simulink model "canard_sim"  (R2026b)
settings: Solver=VariableStepAuto
values from neighbouring files (symbols this model uses):
  boosterCurve = thrustCurve("Data/Cesaroni_2856L910-P.csv")    [TestRocketSetup.m]
  boosterISP = 223    [Full_Rocket_Constants.m]    (also in TestRocketSetup.m = 229)
  InitialMass = SustainerWetMass + BoosterWetMass    (= 57.8)    [Full_Rocket_Constants.m]
  SeparationMass = BoosterDryMass    (= 9.59)    [Full_Rocket_Constants.m]
  stack_t_cg = sus_t_cg(before_sep)    [Full_Rocket_Constants.m]
  stack_x_cg = sus_x_cg(before_sep)    [Full_Rocket_Constants.m]
  Sustainer_Length = 0.381+0.317+1.19    (= 1.888)    [Full_Rocket_Constants.m]
  sustainerISP = 189    [Full_Rocket_Constants.m]
  t_sep = 4.997    [Full_Rocket_Constants.m]
undefined symbols (not defined in the file or in its folder): Stage_Tol, sustainerCurve
libraries: aerolibasang x2, aerolibwind2 x2, aerolibanim x1, aerolibatmos2 x1
settings Model: Creator=linda  LastModifiedBy=linda
settings RTWCC: GPUComputeCapability=5.0

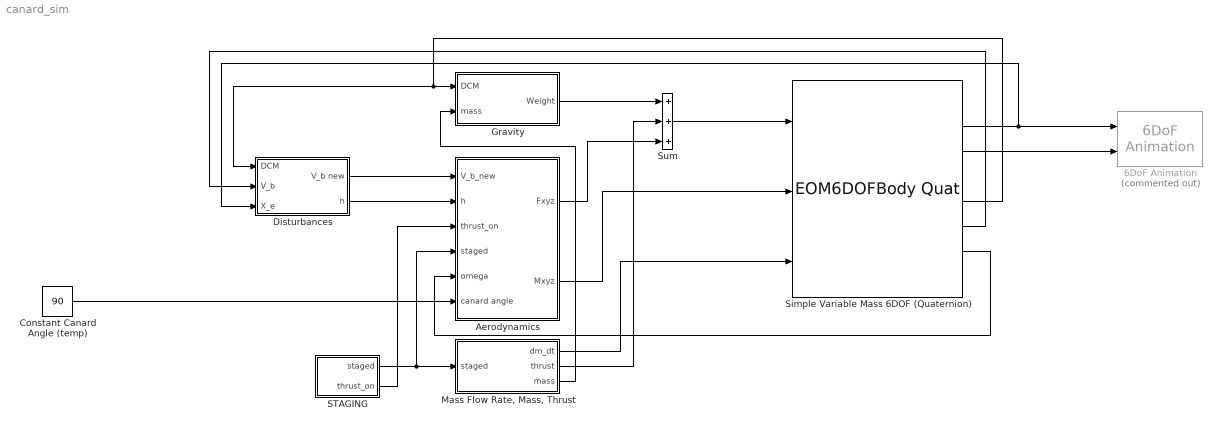
== system canard_sim ==
  6DoF Animation : aerolibanim/6DoF Animation  Commented=on  u1=[-4000 4000 -2000 2000 -5000000 4000000]  u2=0.1  u3=2  u4=[-1000 0 -1000]  u5=Fly alongside  u6=[40 5 -40]  u7=10  u8=on
  Aerodynamics : Subsystem
  Constant Canard Angle (temp) : Constant  Value=90
  Disturbances : Subsystem
  Gravity : Subsystem
  "Mass Flow Rate, Mass, Thrust" : Subsystem
  STAGING : Subsystem
  Simple Variable Mass 6DOF (Quaternion) : EOM6DOFBodyQuat  mtype=Simple Variable
  Sum : Sum  Inputs=+++
  wires:
  Aerodynamics/2(Mxyz) -> Simple Variable Mass 6DOF (Quaternion)/2
  Aerodynamics/1(Fxyz) -> Sum/3
  Sum/1 -> Simple Variable Mass 6DOF (Quaternion)/1
  "Mass Flow Rate, Mass, Thrust"/1(dm_dt) -> Simple Variable Mass 6DOF (Quaternion)/3
  Gravity/1(Weight) -> Sum/1
  "Mass Flow Rate, Mass, Thrust"/2(thrust) -> Sum/2
  Simple Variable Mass 6DOF (Quaternion)/3 -> 6DoF Animation/2
  Simple Variable Mass 6DOF (Quaternion)/2 -> 6DoF Animation/1, Disturbances/3(X_e)
  "Mass Flow Rate, Mass, Thrust"/3(mass) -> Gravity/2(mass)
  Simple Variable Mass 6DOF (Quaternion)/5 -> Disturbances/1(DCM), Gravity/1(DCM)
  Simple Variable Mass 6DOF (Quaternion)/6 -> Disturbances/2(V_b)
  Disturbances/2(h) -> Aerodynamics/2(h)
  STAGING/1(staged) -> "Mass Flow Rate, Mass, Thrust"/1(staged), Aerodynamics/4(staged)
  Disturbances/1(V_b new) -> Aerodynamics/1(V_b_new)
  STAGING/2(thrust_on) -> Aerodynamics/3(thrust_on)
  Simple Variable Mass 6DOF (Quaternion)/7 -> Aerodynamics/5(omega)
  Constant Canard Angle (temp)/1 -> Aerodynamics/6(canard angle)

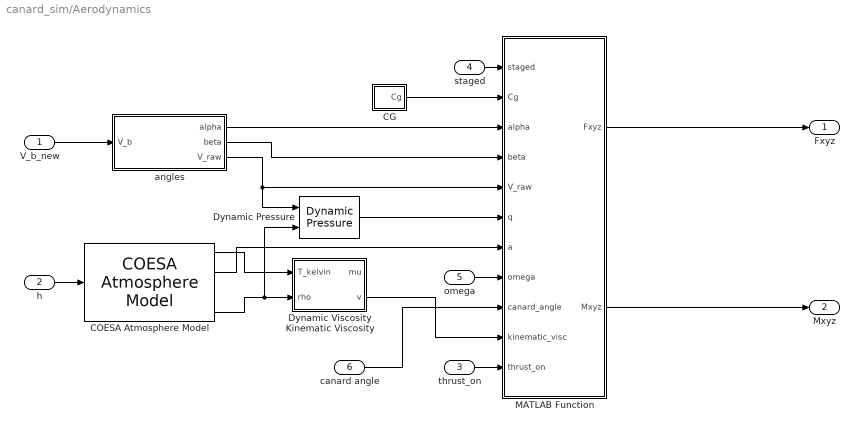
== system canard_sim/Aerodynamics ==
  V_b_new : Inport
  h : Inport  Port=2
  thrust_on : Inport  Port=3
  staged : Inport  Port=4
  omega : Inport  Port=5
  canard angle : Inport  Port=6
  CG : Subsystem
  COESA Atmosphere Model : aerolibatmos2/COESA Atmosphere Model  units=Metric (MKS)  spec=1976 COESA-extended U.S. Standard Atmosphere  model=Profile  profile_var=High temperature  profile_percent=1%  profile_alt=5 km (16404 ft)  envelope_var=High temperature  envelope_percent=1%  action=Warning
  Dynamic Pressure : aerolibasang/Dynamic Pressure
  Dynamic Viscosity Kinematic Viscosity : MATLAB Function  TreatAsAtomicUnit=on
  MATLAB Function : MATLAB Function  TreatAsAtomicUnit=on
  angles : MATLAB Function  TreatAsAtomicUnit=on
  Fxyz : Outport
  Mxyz : Outport  Port=2
  wires:
  COESA Atmosphere Model/1 -> Dynamic Viscosity Kinematic Viscosity/1(T_kelvin)
  COESA Atmosphere Model/4 -> Dynamic Viscosity Kinematic Viscosity/2(rho), Dynamic Pressure/2
  Dynamic Viscosity Kinematic Viscosity/2(v) -> MATLAB Function/10(kinematic_visc)
  Dynamic Pressure/1 -> MATLAB Function/6(q)
  COESA Atmosphere Model/2 -> MATLAB Function/7(a)
  h/1 -> COESA Atmosphere Model/1
  MATLAB Function/1(Fxyz) -> Fxyz/1
  MATLAB Function/2(Mxyz) -> Mxyz/1
  staged/1 -> MATLAB Function/1(staged)
  thrust_on/1 -> MATLAB Function/11(thrust_on)
  omega/1 -> MATLAB Function/8(omega)
  CG/1(Cg) -> MATLAB Function/2(Cg)
  canard angle/1 -> MATLAB Function/9(canard_angle)
  V_b_new/1 -> angles/1(V_b)
  angles/3(V_raw) -> MATLAB Function/5(V_raw), Dynamic Pressure/1
  angles/2(beta) -> MATLAB Function/4(beta)
  angles/1(alpha) -> MATLAB Function/3(alpha)

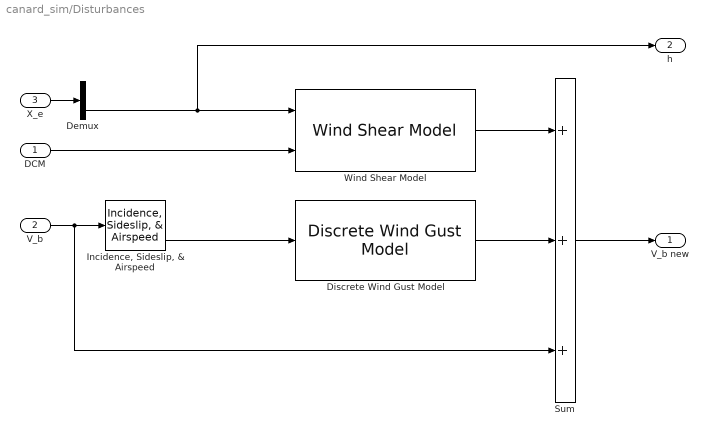
== system canard_sim/Disturbances ==
  DCM : Inport
  V_b : Inport  Port=2
  X_e : Inport  Port=3
  Demux : Demux  Outputs=3
  Discrete Wind Gust Model : aerolibwind2/Discrete Wind Gust Model  units=Metric (MKS)  Gx=on  Gy=on  Gz=on  t_0=5  d_m=[120 120 80]  v_m=[3.5 3.5 3.0]
  "Incidence, Sideslip, & Airspeed" : aerolibasang/Incidence, Sideslip, & Airspeed
  Sum : Sum  Inputs=+++
  Wind Shear Model : aerolibwind2/Wind Shear Model  units=Metric (MKS)  phase=Category C - Terminal Flight Phase  W_20=15  Wdeg=0
  V_b new : Outport
  h : Outport  Port=2
  wires:
  V_b/1 -> Sum/3, "Incidence, Sideslip, & Airspeed"/1
  "Incidence, Sideslip, & Airspeed"/3 -> Discrete Wind Gust Model/1
  Wind Shear Model/1 -> Sum/1
  Discrete Wind Gust Model/1 -> Sum/2
  Sum/1 -> V_b new/1
  DCM/1 -> Wind Shear Model/2
  X_e/1 -> Demux/1
  Demux/3 -> h/1, Wind Shear Model/1

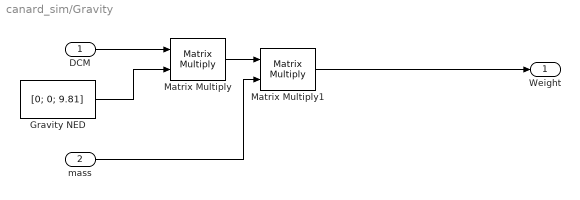
== system canard_sim/Gravity ==
  DCM : Inport
  mass : Inport  Port=2
  Gravity NED : Constant  Value=[0; 0; 9.81]
  Matrix Multiply : Product  Multiplication=Matrix(*)
  Matrix Multiply1 : Product  Multiplication=Matrix(*)
  Weight : Outport
  wires:
  DCM/1 -> Matrix Multiply/1
  Gravity NED/1 -> Matrix Multiply/2
  Matrix Multiply1/1 -> Weight/1
  mass/1 -> Matrix Multiply1/2
  Matrix Multiply/1 -> Matrix Multiply1/1

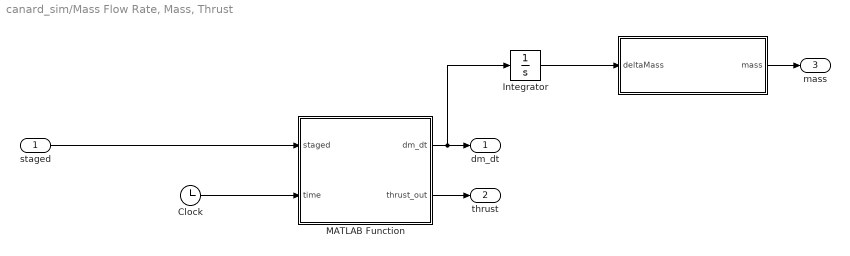
== system canard_sim/Mass Flow Rate, Mass, Thrust ==
  staged : Inport
  " " : MATLAB Function  TreatAsAtomicUnit=on
  Clock : Clock
  Integrator : Integrator
  MATLAB Function : MATLAB Function  TreatAsAtomicUnit=on
  dm_dt : Outport
  thrust : Outport  Port=2
  mass : Outport  Port=3
  wires:
  Clock/1 -> MATLAB Function/2(time)
  staged/1 -> MATLAB Function/1(staged)
  MATLAB Function/1(dm_dt) -> Integrator/1, dm_dt/1
  MATLAB Function/2(thrust_out) -> thrust/1
  Integrator/1 -> " "/1(deltaMass)
  " "/1(mass) -> mass/1

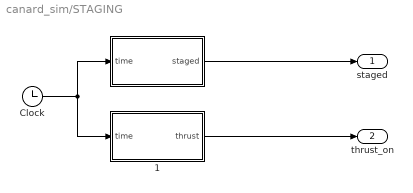
== system canard_sim/STAGING ==
  " " : MATLAB Function  TreatAsAtomicUnit=on
  " 1" : MATLAB Function  TreatAsAtomicUnit=on
  Clock : Clock
  staged : Outport
  thrust_on : Outport  Port=2
  wires:
  " "/1(staged) -> staged/1
  Clock/1 -> " 1"/1(time), " "/1(time)
  " 1"/1(thrust) -> thrust_on/1

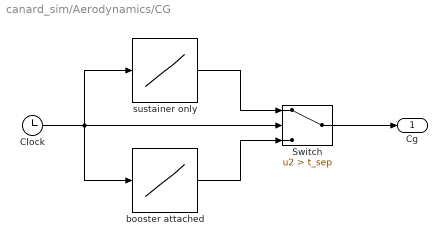
== system canard_sim/Aerodynamics/CG ==
  Clock : Clock
  Switch : Switch  Criteria=u2 > Threshold  Threshold=t_sep  SaturateOnIntegerOverflow=off  InputSameDT=off
  booster attached : Lookup_n-D  NumberOfTableDimensions=1  BreakpointsForDimension1=stack_t_cg  Table=stack_x_cg  ExtrapMethod=Clip  InternalRulePriority=Speed  RndMeth=Simplest
  sustainer only : Lookup_n-D  NumberOfTableDimensions=1  BreakpointsForDimension1=stack_t_cg  Table=stack_x_cg  ExtrapMethod=Clip  InternalRulePriority=Speed  RndMeth=Simplest
  Cg : Outport
  wires:
  Clock/1 -> sustainer only/1, booster attached/1, Switch/2
  Switch/1 -> Cg/1
  booster attached/1 -> Switch/3
  sustainer only/1 -> Switch/1

== matlab function canard_sim/Aerodynamics/MATLAB Function ==
  data: staged input; Fxyz output; Cg input; alpha input; beta input; V_raw input; q input; a input; omega input; canard_angle input; Mxyz output; kinematic_visc input; thrust_on input
function [Fxyz, Mxyz] = aerodynamics(staged, Cg, alpha, beta, V_raw, q, a, omega, canard_angle, kinematic_visc, thrust_on)

== matlab function canard_sim/Aerodynamics/Dynamic Viscosity Kinematic Viscosity ==
  data: T_kelvin input; mu output; rho input; v output
function [mu, v] = fcn(T_kelvin, rho)

% Sutherland's Law

mu_ref = 1.716e-5;  % Pa*s
T_ref = 273.15;     % Kelvin
S = 110.4;          % Kelvin

C1 = (mu_ref*(T_ref+S))/(T_ref^(1.5));

mu = (C1*(T^1.5))/(T_kelvin + S);

v = mu/rho;
;

== matlab function canard_sim/Mass Flow Rate, Mass, Thrust/MATLAB Function ==
  data: dm_dt output; staged input; boosterCurve parameter; sustainerCurve parameter; boosterISP parameter; sustainerISP parameter; time input; Sustainer_Length parameter; Stage_Tol parameter; thrust_out output
function [dm_dt, thrust_out] = mass_flow_rate(staged, boosterCurve, sustainerCurve, boosterISP, sustainerISP, time, Sustainer_Length, Stage_Tol)

g0 = 9.80665;

sustainerIgnitionTime = boosterCurve(end,1) + 2;  % 5.997 s (from openrocket & thrust curves)

% Booster attached
if staged == 0
    thrust = interp1(boosterCurve(:,1), boosterCurve(:,2), time, 'linear', 0);
    dm_dt = -(thrust / (g0 * boosterISP));
% only Sustainer
elseif time >= sustainerIgnitionTime
    sustainerTime = time - sustainerIgnitionTime;

    thrust = interp1(sustainerCurve(:,1), sustainerCurve(:,2), sustainerTime, 'linear', 0);
    dm_dt = -(thrust / (g0 * sustainerISP));
else
    thrust = 0;
    dm_dt = 0;
end

thrust_out = [thrust; 0; 0];  % [Fx; Fy; Fz], N (OR convention)

end

== matlab function canard_sim/Mass Flow Rate, Mass, Thrust/  ==
  data: deltaMass input; mass output; InitialMass parameter; SeparationMass parameter; Sustainer_Length parameter; Stage_Tol parameter
function mass = current_mass(deltaMass, InitialMass, SeparationMass, Sustainer_Length, Stage_Tol)

separated = length <= (Sustainer_Length + Stage_Tol);

mass = InitialMass + deltaMass;

if separated
    mass = mass - SeparationMass;
end
end

== matlab function canard_sim/STAGING/ 1 ==
  data: time input; thrust output
function thrust = thrust_on(time)

if ((boost_start <= time) && (time <= boost_end)) || ((sustain_start <= time) && (time <= sustain_end))
    thrust = 1;
else
    thrust = 0;
end

== matlab function canard_sim/STAGING/  ==
  data: time input; staged output
function staged = staging(time)

if time >= t_sep
    staged = 1;
else
    staged = 0;
end

== matlab function canard_sim/Aerodynamics/angles ==
  data: V_b input; alpha output; beta output; V_raw output
function [alpha, beta, V_raw] = angles(V_b)
